simulink model "flightControlSystem"  (R2026b)
settings: Solver=ode3  StopTime=TFinal
PreLoadFcn:
  | InitVars;
  | definePX4ParamsBus;
undefined symbols (not defined in the file): control_power, DiscIntNeverNeededParam, init, MC_PITCHRATE_MAX, MC_ROLLRATE_MAX, MC_YAWRATE_MAX, PX4_Params_Default, SampleTime, timestamp
libraries: px4Utilslib x52, px4uORBlib x10, vrlib x8, aerolibutil x8, simulink x5, sharedutil x3, matrix_library x2, raspberrypiutilitieslib x2, px4Peripheralslib x2, sharedtransform x1, px4Sensorslib x1
(part 2 of 4)

== system flightControlSystem/MultiCopter Controller/Angular Rate Control/RatePID_Core ==
  note: rate_setpoint = P .* rate_error + rate_int - D .* angular_accel + FF .* rate_sp;
  angular_rate_measured_rads : Inport
  angular_rate_setpoint_rads : Inport  Port=2
  torque_sp_achieved : Inport  Port=3
  vehicle_landed : Inport  Port=4
  mixer_unallocated_torque : Inport  Port=5
  gain_P_MC_ROLLRATE_P : Inport  Port=6
  gain_I_MC_ROLLRATE_I : Inport  Port=7
  gain_D_MC_ROLLRATE_D : Inport  Port=8
  integral_limit_MC_RR_INT_LIM : Inport  Port=9
  dt_s : Inport  Port=10
  angular_accel_filtered_rads2 : Inport  Port=11
  gain_FF_MC_ROLLRATE_FF : Inport  Port=12
  rate_integral_state_prev : Inport  Port=13
  ActuatorSaturation_Detector : Subsystem
  Assignment : Assignment  DiagnosticForDimensions=Warning  IndexOptions=Index vector (dialog)  Indices=3  OutputSizes=1
  DSR_MC_YAW_TQ_CUTOFF : DataStoreRead  DataStoreName=PX4_Params  DataStoreElements=PX4_Params.MC_YAW_TQ_CUTOFF  IndexOptions=Index vector (dialog)  Indices=1  OutputSizes=1
  If_IsLanded : If  IfExpression=u1 ~=0
  Mul_Dterm_D_x_AngAccel : Product
  Mul_FFterm_FF_x_RateSP : Product
  Mul_Pterm_P_x_RateError : Product
  NOT_InvertLanded : Logic  Operator=NOT  IconShape=distinctive  AllPortsSameDT=off  OutDataTypeStr=boolean
  Reshape{1..2,7..11,13} (8 alike) : Reshape
  Selector : Selector  InputPortWidth=3  IndexOptions=Index vector (dialog)  Indices=3  OutputSizes=1
  Sub_RateError_sp_minus_meas : Sum  Inputs=+-
  Sum_PID_FF_TotalTorque : Sum  Inputs=++-+  AccumDataTypeStr=single
  YawTorqueLPF_v116 : MATLAB Function  TreatAsAtomicUnit=on
  rate_integral : Subsystem
  torque_setpoint_Nm : Outport
  rate_integral_state_next : Outport  Port=2
  wires:
  Reshape7/1 -> Mul_Pterm_P_x_RateError/2
  Reshape9/1 -> Mul_Dterm_D_x_AngAccel/1
  gain_FF_MC_ROLLRATE_FF/1 -> Reshape11/1  "ff"
  Mul_Pterm_P_x_RateError/1 -> Sum_PID_FF_TotalTorque/1
  vehicle_landed/1 -> NOT_InvertLanded/1
  angular_rate_setpoint_rads/1 -> Reshape2/1  "rate_sp"
  Sub_RateError_sp_minus_meas/1 -> Reshape7/1, rate_integral/8(rate_error_rads)  "rate_error"
  NOT_InvertLanded/1 -> If_IsLanded/1
  Reshape13/1 -> Sum_PID_FF_TotalTorque/2, rate_integral/9(integral_state_previous)
  Reshape2/1 -> Sub_RateError_sp_minus_meas/1, Mul_FFterm_FF_x_RateSP/2
  angular_rate_measured_rads/1 -> Reshape1/1
  rate_integral_state_prev/1 -> Reshape13/1  "rate_int"
  Reshape11/1 -> Mul_FFterm_FF_x_RateSP/1
  gain_P_MC_ROLLRATE_P/1 -> Reshape8/1  "Prop"
  gain_D_MC_ROLLRATE_D/1 -> Reshape9/1  "Der"
  angular_accel_filtered_rads2/1 -> Reshape10/1  "ang_accel"
  Mul_FFterm_FF_x_RateSP/1 -> Sum_PID_FF_TotalTorque/4
  Reshape8/1 -> Mul_Pterm_P_x_RateError/1
  Reshape10/1 -> Mul_Dterm_D_x_AngAccel/2
  Mul_Dterm_D_x_AngAccel/1 -> Sum_PID_FF_TotalTorque/3
  Reshape1/1 -> Sub_RateError_sp_minus_meas/2
  mixer_unallocated_torque/1 -> ActuatorSaturation_Detector/1(unallocated_torque_3x1)
  torque_sp_achieved/1 -> ActuatorSaturation_Detector/2(torque_setpoint_achieved)
  ActuatorSaturation_Detector/1(is_saturated_positive_3x1) -> rate_integral/1(mixer_saturated_positive)
  ActuatorSaturation_Detector/2(is_saturated_negative_3x1) -> rate_integral/2(mixer_saturated_negative)
  gain_I_MC_ROLLRATE_I/1 -> rate_integral/3(gain_I_per_axis)
  If_IsLanded/1 -> rate_integral/4(landed_reset_to_zero)
  If_IsLanded/2 -> rate_integral/5(airborne_update_integral)
  integral_limit_MC_RR_INT_LIM/1 -> rate_integral/6(integral_limit_symmetric)
  dt_s/1 -> YawTorqueLPF_v116/2(dt), rate_integral/7(dt_s)
  rate_integral/1(integral_state_updated) -> rate_integral_state_next/1
  Sum_PID_FF_TotalTorque/1 -> Selector/1, Assignment/1
  Selector/1 -> YawTorqueLPF_v116/1(yaw_torque)
  YawTorqueLPF_v116/1(yaw_torque_filt) -> Assignment/2
  DSR_MC_YAW_TQ_CUTOFF/1 -> YawTorqueLPF_v116/3(MC_YAW_TQ_CUTOFF)
  Assignment/1 -> torque_setpoint_Nm/1

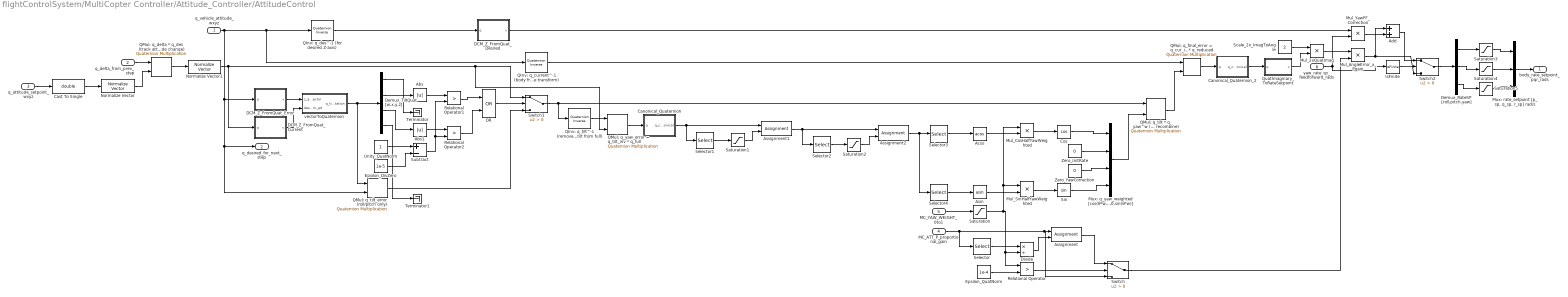
== system flightControlSystem/MultiCopter Controller/Attitude_Controller/AttitudeControl ==
  q_vehicle_attitude_wxyz : Inport
  q_delta_from_prev_step : Inport  Port=2
  q_attitude_setpoint_wxyz : Inport  Port=3
  MC_ATT_P_proportional_gain : Inport  Port=4
  MC_YAW_WEIGHT_0to1 : Inport  Port=5
  yaw_rate_sp_feedforward_rads : Inport  Port=6
  Abs : Abs  SaturateOnIntegerOverflow=off
  Abs1 : Abs  SaturateOnIntegerOverflow=off
  Acos : Trigonometry  Operator=acos
  Add : Sum
  Asin : Trigonometry  Operator=asin
  Assignment : Assignment  DiagnosticForDimensions=Warning  IndexOptions=Index vector (dialog)  Indices=3  OutputSizes=1  RuntimeRangeChecks=off
  Assignment1 : Assignment  DiagnosticForDimensions=Warning  IndexOptions=Index vector (dialog)  Indices=[1]  OutputSizes=1  RuntimeRangeChecks=off
  Assignment2 : Assignment  DiagnosticForDimensions=Warning  IndexOptions=Index vector (dialog)  Indices=[4]  OutputSizes=1  RuntimeRangeChecks=off
  Canonical_Quaternion : MATLAB Function  TreatAsAtomicUnit=on
  Canonical_Quaternion_2 : MATLAB Function  TreatAsAtomicUnit=on
  Cast To Single : DataTypeConversion  OutDataTypeStr=double  SaturateOnIntegerOverflow=off  RndMeth=Floor
  Cos : Trigonometry  Operator=cos
  DCM_Z_FromQuat_Current : MATLAB Function  TreatAsAtomicUnit=on
  DCM_Z_FromQuat_Desired : MATLAB Function  TreatAsAtomicUnit=on
  DCM_Z_FromQuat_Error : MATLAB Function  TreatAsAtomicUnit=on
  Demux_RateSP [roll,pitch,yaw] : Demux  Outputs=3
  Demux_TiltQuat [w,x,y,z] : Demux
  Divide : Product  Inputs=*/
  Epsilon_DivZero : Constant  Value=1e-5  SampleTime=-1
  Epsilon_QuatNorm : Constant  Value=1e-4  OutDataTypeStr=single  SampleTime=-1
  IsFinite : RelationalOperator  Operator=isFinite  OutDataTypeStr=boolean  RndMeth=Simplest  InputSameDT=off
  Mul_2xQuatImag : Product
  Mul_AngleError_x_Pgain : Product
  Mul_CosHalfYawWeighted : Product
  Mul_SinHalfYawWeighted : Product
  Mul_YawFF_Correction : Product
  Mux: q_yaw_weighted [cos(θ*w),0,0,sin(θ*w)] : Mux
  "Mux: rate_setpoint [p_sp, q_sp, r_sp] rad/s" : Mux  Inputs=3
  Normalize Vector : vrlib/Utilities/Normalize Vector  maxzero=0
  Normalize Vector1 : vrlib/Utilities/Normalize Vector  maxzero=0
  OR : Logic  Operator=OR  IconShape=distinctive  AllPortsSameDT=off  OutDataTypeStr=boolean
  QInv: q_current^-1 (body frame transform) : aerolibutil/Quaternion Inverse
  QInv: q_des^-1 (for desired Z-axis) : aerolibutil/Quaternion Inverse
  QInv: q_tilt^-1 (remove tilt from full) : aerolibutil/Quaternion Inverse
  QMul: q_delta * q_des (track attitude change) : aerolibutil/Quaternion Multiplication
  QMul: q_final_error = q_cur_inv * q_reduced : aerolibutil/Quaternion Multiplication
  QMul: q_tilt * q_yaw^w (weighted recombine) : aerolibutil/Quaternion Multiplication
  QMul: q_tilt_error (roll/pitch only) : aerolibutil/Quaternion Multiplication
  QMul: q_yaw_error = q_tilt_inv * q_full : aerolibutil/Quaternion Multiplication
  QuatImaginary_ToRateSetpoint : MATLAB Function  TreatAsAtomicUnit=on
  Relational Operator : RelationalOperator  Operator=>  OutDataTypeStr=boolean  RndMeth=Simplest  InputSameDT=off
  Relational Operator1 : RelationalOperator  Operator=>  OutDataTypeStr=boolean  RndMeth=Simplest  InputSameDT=off
  Relational Operator2 : RelationalOperator  Operator=>  OutDataTypeStr=boolean  RndMeth=Simplest  InputSameDT=off
  Saturation : Saturate  UpperLimit=1  LowerLimit=0
  Saturation1 : Saturate  UpperLimit=1  LowerLimit=-1
  Saturation2 : Saturate  UpperLimit=1  LowerLimit=-1
  Saturation3 : Saturate  UpperLimit=deg2rad(MC_ROLLRATE_MAX)  LowerLimit=-deg2rad(MC_ROLLRATE_MAX)
  Saturation4 : Saturate  UpperLimit=deg2rad(MC_PITCHRATE_MAX)  LowerLimit=-deg2rad(MC_PITCHRATE_MAX)
  Saturation5 : Saturate  UpperLimit=deg2rad(MC_YAWRATE_MAX)  LowerLimit=-deg2rad(MC_YAWRATE_MAX)
  Scale_2x_ImagToAngle : Constant  Value=2  SampleTime=-1
  Selector : Selector  InputPortWidth=3  IndexOptions=Index vector (dialog)  Indices=[3]  OutputSizes=1  RuntimeRangeChecks=off
  Selector1 : Selector  InputPortWidth=4  IndexOptions=Index vector (dialog)  Indices=[1]  OutputSizes=1  RuntimeRangeChecks=off
  Selector2 : Selector  InputPortWidth=4  IndexOptions=Index vector (dialog)  Indices=[4]  OutputSizes=1  RuntimeRangeChecks=off
  Selector3 : Selector  InputPortWidth=4  IndexOptions=Index vector (dialog)  Indices=[1]  OutputSizes=1  RuntimeRangeChecks=off
  Selector4 : Selector  InputPortWidth=4  IndexOptions=Index vector (dialog)  Indices=[4]  OutputSizes=1  RuntimeRangeChecks=off
  Sin : Trigonometry
  Subtract : Sum  Inputs=+-
  Switch : Switch  Criteria=u2 > Threshold  SaturateOnIntegerOverflow=off  InputSameDT=off
  Switch1 : Switch  Criteria=u2 > Threshold  SaturateOnIntegerOverflow=off  InputSameDT=off
  Switch2 : Switch  Criteria=u2 > Threshold  SaturateOnIntegerOverflow=off  InputSameDT=off
  Terminator : Terminator
  Terminator1 : Terminator
  Unity_QuatNorm : Constant  SampleTime=-1
  Zero_InitRate : Constant  Value=0  OutDataTypeStr=single  SampleTime=-1
  Zero_YawCorrection : Constant  Value=0  OutDataTypeStr=single  SampleTime=-1
  vectorToQuaternion : Subsystem
  body_rate_setpoint_pqr_rads : Outport
  q_desired_for_next_step : Outport  Port=2
  wires:
  MC_ATT_P_proportional_gain/1 -> Switch/3, Assignment/1, Selector/1
  Demux_TiltQuat [w,x,y,z]/3 -> Abs1/1
  q_attitude_setpoint_wxyz/1 -> Cast To Single/1
  q_vehicle_attitude_wxyz/1 -> QMul: q_tilt_error (roll/pitch only)/2, q_desired_for_next_step/1, DCM_Z_FromQuat_Error/1(q), QInv: q_current^-1 (body frame transform)/1, QInv: q_des^-1 (for desired Z-axis)/1
  Mul_YawFF_Correction/1 -> Add/2
  Epsilon_DivZero/1 -> Subtract/2
  DCM_Z_FromQuat_Current/1(v) -> vectorToQuaternion/2(desired_z_axis_from_qd)
  q_delta_from_prev_step/1 -> QMul: q_delta * q_des (track attitude change)/1
  Cast To Single/1 -> Normalize Vector/1
  Saturation2/1 -> Assignment2/2
  Switch1/1 -> QMul: q_tilt * q_yaw^w (weighted recombine)/1, QInv: q_tilt^-1 (remove tilt from full)/1
  Normalize Vector/1 -> QMul: q_delta * q_des (track attitude change)/2
  DCM_Z_FromQuat_Desired/1(v) -> Mul_YawFF_Correction/1
  QMul: q_delta * q_des (track attitude change)/1 -> Normalize Vector1/1
  Normalize Vector1/1 -> QMul: q_yaw_error = q_tilt_inv * q_full/2, Switch1/1, DCM_Z_FromQuat_Current/1(q)
  DCM_Z_FromQuat_Error/1(v) -> vectorToQuaternion/1(z_axis_unit_vector)
  QInv: q_des^-1 (for desired Z-axis)/1 -> DCM_Z_FromQuat_Desired/1(q)
  vectorToQuaternion/1(q_tilt_rotation) -> QMul: q_tilt_error (roll/pitch only)/1, Demux_TiltQuat [w,x,y,z]/1
  Demux_TiltQuat [w,x,y,z]/1 -> Terminator/1
  Canonical_Quaternion_2/1(q_canonical) -> QuatImaginary_ToRateSetpoint/1(q)
  Selector3/1 -> Acos/1
  Selector2/1 -> Saturation2/1
  Demux_TiltQuat [w,x,y,z]/2 -> Abs/1
  Demux_TiltQuat [w,x,y,z]/4 -> Terminator1/1
  Epsilon_QuatNorm/1 -> Relational Operator/2
  Unity_QuatNorm/1 -> Subtract/1
  QMul: q_tilt_error (roll/pitch only)/1 -> Switch1/3
  Abs/1 -> Relational Operator1/1
  Mux: q_yaw_weighted [cos(θ*w),0,0,sin(θ*w)]/1 -> QMul: q_tilt * q_yaw^w (weighted recombine)/2
  Relational Operator2/1 -> OR/2
  Abs1/1 -> Relational Operator2/1
  Subtract/1 -> Relational Operator1/2, Relational Operator2/2
  Relational Operator1/1 -> OR/1
  OR/1 -> Switch1/2
  QInv: q_current^-1 (body frame transform)/1 -> QMul: q_final_error = q_cur_inv * q_reduced/1
  QInv: q_tilt^-1 (remove tilt from full)/1 -> QMul: q_yaw_error = q_tilt_inv * q_full/1
  Selector/1 -> Divide/1
  QMul: q_yaw_error = q_tilt_inv * q_full/1 -> Canonical_Quaternion/1(q)
  QMul: q_final_error = q_cur_inv * q_reduced/1 -> Canonical_Quaternion_2/1(q)
  Canonical_Quaternion/1(q_canonical) -> Assignment1/1, Selector1/1
  Selector1/1 -> Saturation1/1
  Cos/1 -> Mux: q_yaw_weighted [cos(θ*w),0,0,sin(θ*w)]/1
  Mul_SinHalfYawWeighted/1 -> Sin/1
  Saturation1/1 -> Assignment1/2
  Assignment1/1 -> Assignment2/1, Selector2/1
  Assignment2/1 -> Selector3/1, Selector4/1
  yaw_rate_sp_feedforward_rads/1 -> IsFinite/1, Mul_YawFF_Correction/2
  Zero_InitRate/1 -> Mux: q_yaw_weighted [cos(θ*w),0,0,sin(θ*w)]/2
  MC_YAW_WEIGHT_0to1/1 -> Saturation/1
  Selector4/1 -> Asin/1
  Acos/1 -> Mul_CosHalfYawWeighted/2
  Assignment/1 -> Switch/1
  Asin/1 -> Mul_SinHalfYawWeighted/2
  Saturation/1 -> Divide/2, Relational Operator/1, Mul_SinHalfYawWeighted/1, Mul_CosHalfYawWeighted/1
  Mul_CosHalfYawWeighted/1 -> Cos/1
  Divide/1 -> Assignment/2
  Relational Operator/1 -> Switch/2
  Sin/1 -> Mux: q_yaw_weighted [cos(θ*w),0,0,sin(θ*w)]/4
  Zero_YawCorrection/1 -> Mux: q_yaw_weighted [cos(θ*w),0,0,sin(θ*w)]/3
  Switch/1 -> Mul_AngleError_x_Pgain/2
  QMul: q_tilt * q_yaw^w (weighted recombine)/1 -> QMul: q_final_error = q_cur_inv * q_reduced/2
  Scale_2x_ImagToAngle/1 -> Mul_2xQuatImag/1
  QuatImaginary_ToRateSetpoint/1(v) -> Mul_2xQuatImag/2
  Mul_2xQuatImag/1 -> Mul_AngleError_x_Pgain/1
  Mul_AngleError_x_Pgain/1 -> Switch2/3, Add/1
  Add/1 -> Switch2/1
  IsFinite/1 -> Switch2/2
  Switch2/1 -> Demux_RateSP [roll,pitch,yaw]/1
  Demux_RateSP [roll,pitch,yaw]/1 -> Saturation3/1
  Demux_RateSP [roll,pitch,yaw]/2 -> Saturation4/1
  Demux_RateSP [roll,pitch,yaw]/3 -> Saturation5/1
  Saturation3/1 -> "Mux: rate_setpoint [p_sp, q_sp, r_sp] rad/s"/1
  Saturation4/1 -> "Mux: rate_setpoint [p_sp, q_sp, r_sp] rad/s"/2
  Saturation5/1 -> "Mux: rate_setpoint [p_sp, q_sp, r_sp] rad/s"/3
  "Mux: rate_setpoint [p_sp, q_sp, r_sp] rad/s"/1 -> body_rate_setpoint_pqr_rads/1

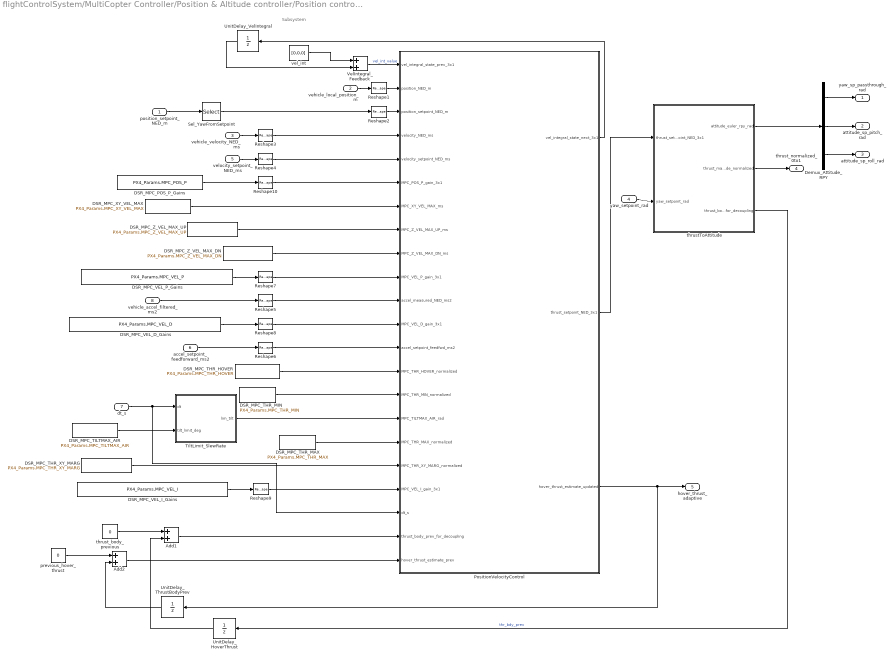
== system flightControlSystem/MultiCopter Controller/Position & Altitude controller/Position controller ==
  note: Subsystem
  position_setpoint_NED_m : Inport
  vehicle_local_position_m : Inport  Port=2
  vehicle_velocity_NED_ms : Inport  Port=3
  yaw_setpoint_rad : Inport  Port=4
  velocity_setpoint_NED_ms : Inport  Port=5
  accel_setpoint_feedforward_ms2 : Inport  Port=6
  dt_s : Inport  Port=7
  vehicle_accel_filtered_ms2 : Inport  Port=8
  Add1 : Sum
  Add2 : Sum
  DSR_MPC_POS_P_Gains : DataStoreRead  DataStoreName=PX4_Params  DataStoreElements=PX4_Params.MPC_POS_P  IndexOptions=Index vector (dialog)  Indices=1  OutputSizes=1
  DSR_MPC_THR_HOVER : DataStoreRead  DataStoreName=PX4_Params  DataStoreElements=PX4_Params.MPC_THR_HOVER  IndexOptions=Index vector (dialog)  Indices=1  OutputSizes=1
  DSR_MPC_THR_MAX : DataStoreRead  DataStoreName=PX4_Params  DataStoreElements=PX4_Params.MPC_THR_MAX  IndexOptions=Index vector (dialog)  Indices=1  OutputSizes=1
  DSR_MPC_THR_MIN : DataStoreRead  DataStoreName=PX4_Params  DataStoreElements=PX4_Params.MPC_THR_MIN  IndexOptions=Index vector (dialog)  Indices=1  OutputSizes=1
  DSR_MPC_THR_XY_MARG : DataStoreRead  DataStoreName=PX4_Params  DataStoreElements=PX4_Params.MPC_THR_XY_MARG  IndexOptions=Index vector (dialog)  Indices=1  OutputSizes=1
  DSR_MPC_TILTMAX_AIR : DataStoreRead  DataStoreName=PX4_Params  DataStoreElements=PX4_Params.MPC_TILTMAX_AIR  IndexOptions=Index vector (dialog)  Indices=1  OutputSizes=1
  DSR_MPC_VEL_D_Gains : DataStoreRead  DataStoreName=PX4_Params  DataStoreElements=PX4_Params.MPC_VEL_D  IndexOptions=Index vector (dialog)  Indices=1  OutputSizes=1
  DSR_MPC_VEL_I_Gains : DataStoreRead  DataStoreName=PX4_Params  DataStoreElements=PX4_Params.MPC_VEL_I  IndexOptions=Index vector (dialog)  Indices=1  OutputSizes=1
  DSR_MPC_VEL_P_Gains : DataStoreRead  DataStoreName=PX4_Params  DataStoreElements=PX4_Params.MPC_VEL_P  IndexOptions=Index vector (dialog)  Indices=1  OutputSizes=1
  DSR_MPC_XY_VEL_MAX : DataStoreRead  DataStoreName=PX4_Params  DataStoreElements=PX4_Params.MPC_XY_VEL_MAX  IndexOptions=Index vector (dialog)  Indices=1  OutputSizes=1
  DSR_MPC_Z_VEL_MAX_DN : DataStoreRead  DataStoreName=PX4_Params  DataStoreElements=PX4_Params.MPC_Z_VEL_MAX_DN  IndexOptions=Index vector (dialog)  Indices=1  OutputSizes=1
  DSR_MPC_Z_VEL_MAX_UP : DataStoreRead  DataStoreName=PX4_Params  DataStoreElements=PX4_Params.MPC_Z_VEL_MAX_UP  IndexOptions=Index vector (dialog)  Indices=1  OutputSizes=1
  Demux_Attitude_RPY : Demux  Outputs=3
  PositionVelocityControl : Subsystem
  Reshape{1..10} (10 alike) : Reshape
  Sel_YawFromSetpoint : Selector  InputPortWidth=4  IndexOptions=Index vector (dialog)  Indices=[1:3]  OutputSizes=1  RuntimeRangeChecks=off
  TiltLimit_SlewRate : MATLAB Function  TreatAsAtomicUnit=on
  UnitDelay_HoverThrust : UnitDelay  SampleTime=-1
  UnitDelay_ThrustBodyPrev : UnitDelay  SampleTime=-1
  UnitDelay_VelIntegral : UnitDelay  InitialCondition=[0; 0; 0]  SampleTime=-1
  VelIntegral_Feedback : Sum
  previous_hover_thrust : Constant  Value=0  OutDataTypeStr=single  SampleTime=-1
  thrustToAttitude : Subsystem
  thrust_body_previous : Constant  Value=0  OutDataTypeStr=single  SampleTime=-1
  vel_int : Constant  Value=[0,0,0]  OutDataTypeStr=single  SampleTime=-1
  yaw_sp_passthrough_rad : Outport
  attitude_sp_pitch_rad : Outport  Port=2
  attitude_sp_roll_rad : Outport  Port=3
  thrust_normalized_0to1 : Outport  Port=4
  hover_thrust_adaptive : Outport  Port=5
  wires:
  thrustToAttitude/1(attitude_euler_rpy_rad) -> Demux_Attitude_RPY/1
  previous_hover_thrust/1 -> Add2/1
  vel_int/1 -> VelIntegral_Feedback/1
  thrust_body_previous/1 -> Add1/1
  position_setpoint_NED_m/1 -> Sel_YawFromSetpoint/1
  UnitDelay_HoverThrust/1 -> Add1/2
  DSR_MPC_TILTMAX_AIR/1 -> TiltLimit_SlewRate/2(tilt_limit_deg)
  UnitDelay_VelIntegral/1 -> VelIntegral_Feedback/2
  UnitDelay_ThrustBodyPrev/1 -> Add2/2
  Demux_Attitude_RPY/1 -> yaw_sp_passthrough_rad/1
  thrustToAttitude/2(thrust_magnitude_normalized) -> thrust_normalized_0to1/1
  PositionVelocityControl/3(hover_thrust_estimate_updated) -> UnitDelay_ThrustBodyPrev/1, hover_thrust_adaptive/1
  PositionVelocityControl/1(vel_integral_state_next_3x1) -> UnitDelay_VelIntegral/1
  Demux_Attitude_RPY/3 -> attitude_sp_roll_rad/1
  Demux_Attitude_RPY/2 -> attitude_sp_pitch_rad/1
  thrustToAttitude/3(thrust_body_frame_for_decoupling) -> UnitDelay_HoverThrust/1  "thr_bdy_prev"
  PositionVelocityControl/2(thrust_setpoint_NED_3x1) -> thrustToAttitude/1(thrust_setpoint_NED_3x1)
  Reshape9/1 -> PositionVelocityControl/19(MPC_VEL_I_gain_3x1)
  DSR_MPC_THR_XY_MARG/1 -> PositionVelocityControl/18(MPC_THR_XY_MARG_normalized)
  DSR_MPC_THR_MAX/1 -> PositionVelocityControl/17(MPC_THR_MAX_normalized)
  dt_s/1 -> TiltLimit_SlewRate/1(dt), PositionVelocityControl/20(dt_s)
  DSR_MPC_THR_MIN/1 -> PositionVelocityControl/15(MPC_THR_MIN_normalized)
  DSR_MPC_THR_HOVER/1 -> PositionVelocityControl/14(MPC_THR_HOVER_normalized)
  Reshape6/1 -> PositionVelocityControl/13(accel_setpoint_feedfwd_ms2)
  Reshape8/1 -> PositionVelocityControl/12(MPC_VEL_D_gain_3x1)
  Reshape7/1 -> PositionVelocityControl/10(MPC_VEL_P_gain_3x1)
  DSR_MPC_Z_VEL_MAX_UP/1 -> PositionVelocityControl/8(MPC_Z_VEL_MAX_UP_ms)
  Reshape10/1 -> PositionVelocityControl/6(MPC_POS_P_gain_3x1)
  Reshape4/1 -> PositionVelocityControl/5(velocity_setpoint_NED_ms)
  Reshape5/1 -> PositionVelocityControl/11(accel_measured_NED_ms2)
  Reshape3/1 -> PositionVelocityControl/4(velocity_NED_ms)
  Reshape2/1 -> PositionVelocityControl/3(position_setpoint_NED_m)
  accel_setpoint_feedforward_ms2/1 -> Reshape6/1
  DSR_MPC_XY_VEL_MAX/1 -> PositionVelocityControl/7(MPC_XY_VEL_MAX_ms)
  DSR_MPC_VEL_P_Gains/1 -> Reshape7/1
  yaw_setpoint_rad/1 -> thrustToAttitude/2(yaw_setpoint_rad)
  DSR_MPC_POS_P_Gains/1 -> Reshape10/1
  Reshape1/1 -> PositionVelocityControl/2(position_NED_m)
  DSR_MPC_Z_VEL_MAX_DN/1 -> PositionVelocityControl/9(MPC_Z_VEL_MAX_DN_ms)
  vehicle_accel_filtered_ms2/1 -> Reshape5/1
  velocity_setpoint_NED_ms/1 -> Reshape4/1
  vehicle_velocity_NED_ms/1 -> Reshape3/1
  Sel_YawFromSetpoint/1 -> Reshape2/1
  vehicle_local_position_m/1 -> Reshape1/1
  DSR_MPC_VEL_D_Gains/1 -> Reshape8/1
  DSR_MPC_VEL_I_Gains/1 -> Reshape9/1
  TiltLimit_SlewRate/1(lim_tilt) -> PositionVelocityControl/16(MPC_TILTMAX_AIR_rad)
  VelIntegral_Feedback/1 -> PositionVelocityControl/1(vel_integral_state_prev_3x1)  "vel_int_value"
  Add1/1 -> PositionVelocityControl/21(thrust_body_prev_for_decoupling)
  Add2/1 -> PositionVelocityControl/22(hover_thrust_estimate_prev)

== system flightControlSystem/ParamUpdate/HW_ParamUpdate/ReadParams_OnUpdate ==
  Enable : EnablePort
  AttitudeCtrl_Params : Subsystem
  BusCreator_Params : BusCreator  Inputs=30  OutDataTypeStr=Bus: PX4_Params_Bus
  Estimator_Params : Subsystem
  LandingLogic_Params : Subsystem
  PositionCtrl_Params : Subsystem
  RateCtrl_Params : Subsystem
  Signal Conversion : SignalConversion  ConversionOutput=Nonvirtual bus  OverrideOpt=off
  Write_PX4_Params : DataStoreWrite  DataStoreName=PX4_Params  IndexOptions=Index vector (dialog)  Indices=1  OutputSizes=1
  wires:
  RateCtrl_Params/4(MC_RATE_FF) -> BusCreator_Params/19  "MC_RATE_FF"
  PositionCtrl_Params/8(MPC_THR_XY_MARG) -> BusCreator_Params/8  "MPC_THR_XY_MARG"
  Estimator_Params/2(EST_NF_FRQ) -> BusCreator_Params/29  "EST_NF_FRQ"
  LandingLogic_Params/6(MPC_Z_VEL_MAX_DN_LAND) -> BusCreator_Params/27  "MPC_Z_VEL_MAX_DN_LAND"
  PositionCtrl_Params/2(MPC_VEL_P) -> BusCreator_Params/2  "MPC_VEL_P"
  PositionCtrl_Params/1(MPC_POS_P) -> BusCreator_Params/1  "MPC_POS_P"
  PositionCtrl_Params/5(MPC_THR_HOVER) -> BusCreator_Params/5  "MPC_THR_HOVER"
  PositionCtrl_Params/11(MPC_Z_VEL_MAX_UP) -> BusCreator_Params/11  "MPC_Z_VEL_MAX_UP"
  Estimator_Params/1(MPC_VELD_LP) -> BusCreator_Params/28  "MPC_VELD_LP"
  AttitudeCtrl_Params/2(MC_YAW_WEIGHT) -> BusCreator_Params/15  "MC_YAW_WEIGHT"
  PositionCtrl_Params/3(MPC_VEL_I) -> BusCreator_Params/3  "MPC_VEL_I"
  PositionCtrl_Params/6(MPC_THR_MAX) -> BusCreator_Params/6  "MPC_THR_MAX"
  Estimator_Params/3(EST_NF_BW) -> BusCreator_Params/30  "EST_NF_BW"
  Signal Conversion/1 -> Write_PX4_Params/1
  PositionCtrl_Params/4(MPC_VEL_D) -> BusCreator_Params/4  "MPC_VEL_D"
  BusCreator_Params/1 -> Signal Conversion/1
  LandingLogic_Params/1(MPC_LAND_ALT1) -> BusCreator_Params/22  "MPC_LAND_ALT1"
  LandingLogic_Params/2(MPC_LAND_ALT2) -> BusCreator_Params/23  "MPC_LAND_ALT2"
  PositionCtrl_Params/7(MPC_THR_MIN) -> BusCreator_Params/7  "MPC_THR_MIN"
  AttitudeCtrl_Params/1(MC_ATT_P) -> BusCreator_Params/14  "MC_ATT_P"
  LandingLogic_Params/3(MPC_LAND_ALT3) -> BusCreator_Params/24  "MPC_LAND_ALT3"
  RateCtrl_Params/2(MC_RATE_I) -> BusCreator_Params/17  "MC_RATE_I"
  LandingLogic_Params/4(MPC_LAND_SPEED) -> BusCreator_Params/25  "MPC_LAND_SPEED"
  LandingLogic_Params/5(MPC_LAND_CRWL) -> BusCreator_Params/26  "MPC_LAND_CRWL"
  PositionCtrl_Params/9(MPC_TILTMAX_AIR) -> BusCreator_Params/9  "MPC_TILTMAX_AIR"
  RateCtrl_Params/5(MC_RATE_INT_LIM) -> BusCreator_Params/20  "MC_RATE_INT_LIM"
  RateCtrl_Params/1(MC_RATE_P) -> BusCreator_Params/16  "MC_RATE_P"
  RateCtrl_Params/6(MC_YAW_TQ_CUTOFF) -> BusCreator_Params/21  "MC_YAW_TQ_CUTOFF"
  PositionCtrl_Params/10(MPC_XY_VEL_MAX) -> BusCreator_Params/10  "MPC_XY_VEL_MAX"
  PositionCtrl_Params/12(MPC_Z_VEL_MAX_DN) -> BusCreator_Params/12  "MPC_Z_VEL_MAX_DN"
  RateCtrl_Params/3(MC_RATE_D) -> BusCreator_Params/18  "MC_RATE_D"
  PositionCtrl_Params/13(MPC_ACC_DECOUPLE) -> BusCreator_Params/13  "MPC_ACC_DECOUPLE"

== system flightControlSystem/SetpointManager/Set target Position/Landing Logic ==
  Current_Pos : Inport
  land_trigger : Inport  Port=2
  DSR_MPC_LAND_ALT1 : DataStoreRead  DataStoreName=PX4_Params  DataStoreElements=PX4_Params.MPC_LAND_ALT1  IndexOptions=Index vector (dialog)  Indices=1  OutputSizes=1
  DSR_MPC_LAND_ALT2 : DataStoreRead  DataStoreName=PX4_Params  DataStoreElements=PX4_Params.MPC_LAND_ALT2  IndexOptions=Index vector (dialog)  Indices=1  OutputSizes=1
  DSR_MPC_LAND_ALT3 : DataStoreRead  DataStoreName=PX4_Params  DataStoreElements=PX4_Params.MPC_LAND_ALT3  IndexOptions=Index vector (dialog)  Indices=1  OutputSizes=1
  DSR_MPC_LAND_CRWL : DataStoreRead  DataStoreName=PX4_Params  DataStoreElements=PX4_Params.MPC_LAND_CRWL  IndexOptions=Index vector (dialog)  Indices=1  OutputSizes=1
  DSR_MPC_LAND_SPEED : DataStoreRead  DataStoreName=PX4_Params  DataStoreElements=PX4_Params.MPC_LAND_SPEED  IndexOptions=Index vector (dialog)  Indices=1  OutputSizes=1
  DSR_MPC_Z_VEL_MAX_DN : DataStoreRead  DataStoreName=PX4_Params  DataStoreElements=PX4_Params.MPC_Z_VEL_MAX_DN_LAND  IndexOptions=Index vector (dialog)  Indices=1  OutputSizes=1
  PX4 Landing Logic : MATLAB Function  TreatAsAtomicUnit=on
  Selector1 : Selector  InputPortWidth=5  IndexOptions=Index vector (dialog)  Indices=[1:4]  OutputSizes=1  RuntimeRangeChecks=off
  pos_sp : Outport
  vel_sp : Outport  Port=2
  acc_sp : Outport  Port=3
  wires:
  Current_Pos/1 -> Selector1/1
  DSR_MPC_LAND_CRWL/1 -> PX4 Landing Logic/4(MPC_LAND_CRWL_in)
  Selector1/1 -> PX4 Landing Logic/2(states)
  DSR_MPC_LAND_SPEED/1 -> PX4 Landing Logic/3(MPC_LAND_SPEED_in)
  DSR_MPC_LAND_ALT1/1 -> PX4 Landing Logic/5(MPC_LAND_ALT1_in)
  DSR_MPC_Z_VEL_MAX_DN/1 -> PX4 Landing Logic/8(MPC_Z_VEL_MAX_DN_in)
  DSR_MPC_LAND_ALT2/1 -> PX4 Landing Logic/6(MPC_LAND_ALT2_in)
  DSR_MPC_LAND_ALT3/1 -> PX4 Landing Logic/7(MPC_LAND_ALT3_in)
  PX4 Landing Logic/1(pos_sp) -> pos_sp/1
  PX4 Landing Logic/2(vel_sp) -> vel_sp/1
  PX4 Landing Logic/3(acc_sp) -> acc_sp/1
  land_trigger/1 -> PX4 Landing Logic/1(land_trigger)

== system flightControlSystem/SetpointManager/Set target Position/Logger ==
  DesiredPosition : Inport
  DesiredVelocity : Inport  Port=2
  DesiredAcceleration : Inport  Port=3
  States : Inport  Port=4
  Cast To Single{,1..13} (14 alike) : DataTypeConversion  OutDataTypeStr=single  SaturateOnIntegerOverflow=off  RndMeth=Floor
  Demux : Demux
  Demux1 : Demux
  Demux2 : Demux  Outputs=3
  Demux3 : Demux  Outputs=3
  PX4 ULog : px4Utilslib/PX4 ULog  Commented=on  uORBMsg=FlightChecks
  Rate Transition : RateTransition
  Rate Transition2 : RateTransition
  Selector : Selector  InputPortWidth=5  IndexOptions=Index vector (dialog)  Indices=[1:4]  OutputSizes=1
  wires:
  Cast To Single2/1 -> ?
  Demux/1 -> Cast To Single/1
  Cast To Single5/1 -> PX4 ULog/2
  Rate Transition2/1 -> Demux1/1
  Demux1/3 -> Cast To Single6/1
  Cast To Single7/1 -> PX4 ULog/4
  Demux1/1 -> Cast To Single4/1
  Rate Transition/1 -> Demux/1
  Cast To Single6/1 -> PX4 ULog/3
  DesiredPosition/1 -> Rate Transition2/1
  DesiredAcceleration/1 -> Demux3/1
  Demux1/2 -> Cast To Single5/1
  Demux2/1 -> Cast To Single8/1
  Cast To Single4/1 -> PX4 ULog/1
  Demux3/2 -> Cast To Single12/1
  Demux/2 -> Cast To Single1/1
  Demux1/4 -> Cast To Single7/1
  Cast To Single8/1 -> ?
  Demux2/2 -> Cast To Single9/1
  Cast To Single9/1 -> ?
  Cast To Single10/1 -> ?
  Demux2/3 -> Cast To Single10/1
  Demux3/1 -> Cast To Single11/1
  Cast To Single11/1 -> ?
  Cast To Single13/1 -> ?
  Cast To Single12/1 -> ?
  Demux3/3 -> Cast To Single13/1
  Cast To Single/1 -> ?
  Cast To Single1/1 -> ?
  Demux/3 -> Cast To Single2/1
  Demux/4 -> Cast To Single3/1
  Cast To Single3/1 -> ?
  States/1 -> Selector/1
  DesiredVelocity/1 -> Demux2/1
  Selector/1 -> Rate Transition/1

== system flightControlSystem/SetpointManager/Set target Position/RC Failsafe Signal ==
  note: Channel 7 - RC Flysky
      | Channel 7 - Dexi Radiomaster
  Constant1 : Constant  SampleTime=-1
  MATLAB Function : MATLAB Function  TreatAsAtomicUnit=on
  Radio Control Transmitter1 : px4Sensorslib/Radio Control Transmitter  channel1=off  channel2=off  channel3=off  channel4=off  channel5=off  channel6=off  channel7=on  channel8=off  channel_count=off  rssi=on  rc_input_source=off  timestamp_last_signal=off  time_stamp=off  sampleTime=1/250  BlockingMode=off  BlockTimeout=5
  Rate Transition3 : RateTransition
  Switch1 : Switch  Criteria=u2 ~= 0  SaturateOnIntegerOverflow=off  InputSameDT=off
  Unit Delay : UnitDelay  SampleTime=-1
  Land_Trigger : Outport
  wires:
  Constant1/1 -> Switch1/1
  Radio Control Transmitter1/3 -> MATLAB Function/3(RSSI)
  Radio Control Transmitter1/2 -> MATLAB Function/2(ch7)
  Radio Control Transmitter1/1 -> MATLAB Function/1(status)
  MATLAB Function/1(out) -> Rate Transition3/1
  Rate Transition3/1 -> Switch1/2
  Unit Delay/1 -> Switch1/3
  Switch1/1 -> Unit Delay/1, Land_Trigger/1

== system flightControlSystem/SetpointManager/Set target Position/Setpoints Selector ==
  Land_Pos : Inport
  Land_Vel : Inport  Port=2
  Land_Acc : Inport  Port=3
  LandTrigger : Inport  Port=4
  Des_Pos : Inport  Port=5
  Des_Vel : Inport  Port=6
  Des_Acc : Inport  Port=7
  Acc Switch : Switch  Criteria=u2 > Threshold  SaturateOnIntegerOverflow=off  InputSameDT=off
  Rate Transition2 : RateTransition
  Rate Transition4 : RateTransition
  Rate Transition5 : RateTransition
  Reshape : Reshape
  Switch : Switch  Criteria=u2 > Threshold  SaturateOnIntegerOverflow=off  InputSameDT=off
  Vel Switch : Switch  Criteria=u2 > Threshold  SaturateOnIntegerOverflow=off  InputSameDT=off
  des_pos : Outport
  des_vel : Outport  Port=2
  des_acc : Outport  Port=3
  wires:
  Land_Acc/1 -> Acc Switch/1
  Acc Switch/1 -> Rate Transition5/1
  Reshape/1 -> Switch/1
  LandTrigger/1 -> Vel Switch/2, Switch/2, Acc Switch/2
  Switch/1 -> Rate Transition2/1
  Vel Switch/1 -> Rate Transition4/1
  Land_Pos/1 -> Reshape/1
  Land_Vel/1 -> Vel Switch/1
  Rate Transition2/1 -> des_pos/1
  Des_Pos/1 -> Switch/3
  Rate Transition4/1 -> des_vel/1
  Des_Vel/1 -> Vel Switch/3
  Rate Transition5/1 -> des_acc/1
  Des_Acc/1 -> Acc Switch/3

== system flightControlSystem/SetpointManager/Set target Position/Setpoints from Perception Module ==
  CurrentPosition : Inport
  AND : Logic  IconShape=distinctive  AllPortsSameDT=off  OutDataTypeStr=boolean
  Cast To Boolean : DataTypeConversion  OutDataTypeStr=boolean  SaturateOnIntegerOverflow=off  RndMeth=Floor
  Cast To Double : DataTypeConversion  OutDataTypeStr=double  SaturateOnIntegerOverflow=off  RndMeth=Floor
  Compare To Constant1 : simulink/Logic and Bit Operations/Compare To Constant  relop===  const=222  OutDataTypeStr=boolean
  Demux : Demux  Outputs=11
  Enabled Subsystem : Subsystem  TreatAsAtomicUnit=on
  Mux : Mux
  Mux1 : Mux  Inputs=3
  Mux2 : Mux  Inputs=3
  Protocol Decoder : raspberrypiutilitieslib/Protocol Decoder  IsParseCSV=off  Header=[134]  FieldTable={ 'Field1', '11', 'single', 'Little endian' }  IsVariableSizeLastField=off  MaxVariableSizeFieldLength=[]  IsChecksumRequired=off  ChecksumAlgorithm=XOR of bytes  ChecksumSize=[]  TerminatorOption=<none>  CustomTerminatorVal=[]  IsInputLengthAvailable=off
  Selector : Selector  InputPortWidth=5  IndexOptions=Index vector (dialog)  Indices=[5]  OutputSizes=1  RuntimeRangeChecks=off
  Serial Receive : px4Peripheralslib/Serial Receive  SCIModule=/dev/ttyACM0  DataType=uint8  DataLength=45  OutputStatus=on  SampleTime=1/10  BlockingMode=off  PartialData=on  Timeout=5
  Switch2 : Switch  Criteria=u2 > Threshold  SaturateOnIntegerOverflow=off  InputSameDT=off
  Terminator : Terminator
  Terminator1 : Terminator
  Unit Delay : UnitDelay  SampleTime=-1
  des Position : Outport
  desired Velocity : Outport  Port=2
  desired Acceleration : Outport  Port=3
  wires:
  Demux/1 -> Mux/1
  Demux/3 -> Mux/3
  Demux/11 -> Compare To Constant1/1
  AND/1 -> Enabled Subsystem/Enable
  Demux/6 -> Mux1/2
  Demux/10 -> Mux2/3
  Selector/1 -> Cast To Boolean/1
  Compare To Constant1/1 -> AND/2, Switch2/2
  Protocol Decoder/1 -> Cast To Double/1
  Cast To Double/1 -> Demux/1
  Demux/2 -> Mux/2
  Demux/9 -> Mux2/2
  Protocol Decoder/2 -> Terminator/1
  Cast To Boolean/1 -> AND/1
  Demux/8 -> Mux2/1
  Demux/5 -> Mux1/1
  Serial Receive/1 -> Protocol Decoder/1
  Mux/1 -> Switch2/1
  Unit Delay/1 -> Switch2/3
  Switch2/1 -> des Position/1, Unit Delay/1
  CurrentPosition/1 -> Selector/1, Enabled Subsystem/1(CurrentPosition)
  Demux/4 -> Mux/4
  Demux/7 -> Mux1/3
  Serial Receive/2 -> Terminator1/1
  Mux1/1 -> desired Velocity/1
  Mux2/1 -> desired Acceleration/1

== system flightControlSystem/SetpointManager/Simulation Set target Position/Landing Logic ==
  Current_Pos : Inport
  land_trigger : Inport  Port=2
  DSR_MPC_LAND_ALT1_const : DataStoreRead  DataStoreName=PX4_Params  DataStoreElements=PX4_Params.MPC_LAND_ALT1  IndexOptions=Index vector (dialog)  Indices=1  OutputSizes=1
  DSR_MPC_LAND_ALT2_const : DataStoreRead  DataStoreName=PX4_Params  DataStoreElements=PX4_Params.MPC_LAND_ALT2  IndexOptions=Index vector (dialog)  Indices=1  OutputSizes=1
  DSR_MPC_LAND_ALT3_const : DataStoreRead  DataStoreName=PX4_Params  DataStoreElements=PX4_Params.MPC_LAND_ALT3  IndexOptions=Index vector (dialog)  Indices=1  OutputSizes=1
  DSR_MPC_LAND_CRWL_const : DataStoreRead  DataStoreName=PX4_Params  DataStoreElements=PX4_Params.MPC_LAND_CRWL  IndexOptions=Index vector (dialog)  Indices=1  OutputSizes=1
  DSR_MPC_LAND_SPEED_const : DataStoreRead  DataStoreName=PX4_Params  DataStoreElements=PX4_Params.MPC_LAND_SPEED  IndexOptions=Index vector (dialog)  Indices=1  OutputSizes=1
  DSR_MPC_Z_VEL_MAX_DN_const : DataStoreRead  DataStoreName=PX4_Params  DataStoreElements=PX4_Params.MPC_Z_VEL_MAX_DN_LAND  IndexOptions=Index vector (dialog)  Indices=1  OutputSizes=1
  PX4 Landing Logic : MATLAB Function  TreatAsAtomicUnit=on
  Selector1 : Selector  InputPortWidth=5  IndexOptions=Index vector (dialog)  Indices=[1:4]  OutputSizes=1  RuntimeRangeChecks=off
  pos_sp : Outport
  vel_sp : Outport  Port=2
  acc_sp : Outport  Port=3
  wires:
  Current_Pos/1 -> Selector1/1
  DSR_MPC_LAND_CRWL_const/1 -> PX4 Landing Logic/4(MPC_LAND_CRWL_in)
  Selector1/1 -> PX4 Landing Logic/2(states)
  DSR_MPC_LAND_SPEED_const/1 -> PX4 Landing Logic/3(MPC_LAND_SPEED_in)
  DSR_MPC_LAND_ALT1_const/1 -> PX4 Landing Logic/5(MPC_LAND_ALT1_in)
  DSR_MPC_Z_VEL_MAX_DN_const/1 -> PX4 Landing Logic/8(MPC_Z_VEL_MAX_DN_in)
  DSR_MPC_LAND_ALT2_const/1 -> PX4 Landing Logic/6(MPC_LAND_ALT2_in)
  DSR_MPC_LAND_ALT3_const/1 -> PX4 Landing Logic/7(MPC_LAND_ALT3_in)
  PX4 Landing Logic/1(pos_sp) -> pos_sp/1
  PX4 Landing Logic/2(vel_sp) -> vel_sp/1
  PX4 Landing Logic/3(acc_sp) -> acc_sp/1
  land_trigger/1 -> PX4 Landing Logic/1(land_trigger)

== system flightControlSystem/SetpointManager/Simulation Set target Position/Setpoints Selector ==
  Land_Pos : Inport
  Land_Vel : Inport  Port=2
  Land_Acc : Inport  Port=3
  LandTrigger : Inport  Port=4
  Des_Pos : Inport  Port=5
  Des_Vel : Inport  Port=6
  Des_Acc : Inport  Port=7
  Acc Switch : Switch  Criteria=u2 > Threshold  SaturateOnIntegerOverflow=off  InputSameDT=off
  Rate Transition2 : RateTransition
  Rate Transition4 : RateTransition
  Rate Transition5 : RateTransition
  Reshape : Reshape
  Switch : Switch  Criteria=u2 > Threshold  SaturateOnIntegerOverflow=off  InputSameDT=off
  Vel Switch : Switch  Criteria=u2 > Threshold  SaturateOnIntegerOverflow=off  InputSameDT=off
  des_pos : Outport
  des_vel : Outport  Port=2
  des_acc : Outport  Port=3
  wires:
  Land_Acc/1 -> Acc Switch/1
  Acc Switch/1 -> Rate Transition5/1
  Reshape/1 -> Switch/1
  LandTrigger/1 -> Vel Switch/2, Switch/2, Acc Switch/2
  Switch/1 -> Rate Transition2/1
  Vel Switch/1 -> Rate Transition4/1
  Land_Pos/1 -> Reshape/1
  Land_Vel/1 -> Vel Switch/1
  Rate Transition2/1 -> des_pos/1
  Des_Pos/1 -> Switch/3
  Rate Transition4/1 -> des_vel/1
  Des_Vel/1 -> Vel Switch/3
  Rate Transition5/1 -> des_acc/1
  Des_Acc/1 -> Acc Switch/3

== system flightControlSystem/Actuator Commands/Simulation Actuator Commands/Mixer/Battery_Scaling ==
  In1 : Inport
  In2 : Inport  Port=2
  Compare To Constant : simulink/Logic and Bit Operations/Compare To Constant  relop=~=  const=0  OutDataTypeStr=boolean
  Constant : Constant  SampleTime=SampleTime
  Demux1 : Demux  Outputs=3
  Gain : Gain  Gain=-1
  Product : Product
  Product2 : Product
  Saturation1 : Saturate  UpperLimit=1  LowerLimit=-1
  Saturation2 : Saturate  UpperLimit=1  LowerLimit=-1
  Switch : Switch  Criteria=u2 > Threshold  SaturateOnIntegerOverflow=off  InputSameDT=off
  Switch1 : Switch  Criteria=u2 > Threshold  SaturateOnIntegerOverflow=off  InputSameDT=off
  thrust_setpoint : Outport
  pitch : Outport  Port=2
  roll : Outport  Port=3
  yaw : Outport  Port=4
  wires:
  Constant/1 -> Product2/2, Compare To Constant/1, Product/2  "<scale>"
  In1/1 -> Switch/3, Product/1
  In2/1 -> Switch1/3, Product2/1
  Switch/1 -> Gain/1
  Product/1 -> Switch/1
  Gain/1 -> Saturation2/1
  Demux1/3 -> yaw/1
  Switch1/1 -> Saturation1/1
  Compare To Constant/1 -> Switch1/2, Switch/2
  Saturation1/1 -> Demux1/1  "torque_setpoint"
  Product2/1 -> Switch1/1
  Demux1/1 -> roll/1
  Demux1/2 -> pitch/1
  Saturation2/1 -> thrust_setpoint/1  "thrust_setpoint"

== system flightControlSystem/MultiCopter Controller/Angular Rate Control/RateIntegral_State/Set target Position ==
  Control_Power : Inport
  Bus Assignment : BusAssignment  AssignedSignals=timestamp,control_power
  PX4 Timestamp : px4Utilslib/PX4 Timestamp  SampleTime=-1
  PX4 uORB Message : px4uORBlib/PX4 uORB Message  uORBMsg=ActuatorControlsStatus  uORBTopicName=actuator_controls_status_0  isSingleTopicMsg=off  SampleTime=-1
  PX4 uORB Write : px4uORBlib/PX4 uORB Write  uORBMsg=ActuatorControlsStatus  uORBTopicName=actuator_controls_status_0  PublishOption=None  OutputPublishedInstanceNum=off  selectInstanceNum=1  OutputStatus=off  isSingleTopicMsg=off
  wires:
  PX4 Timestamp/1 -> Bus Assignment/2
  PX4 uORB Message/1 -> Bus Assignment/1
  Bus Assignment/1 -> PX4 uORB Write/1
  Control_Power/1 -> Bus Assignment/3

== system flightControlSystem/MultiCopter Controller/Angular Rate Control/RateIntegral_State/Simulation Set target Position ==
  Control_Power : Inport
  Terminator3 : Terminator
  wires:
  Control_Power/1 -> Terminator3/1

== system flightControlSystem/MultiCopter Controller/Angular Rate Control/RatePID_Core/ActuatorSaturation_Detector ==
  unallocated_torque_3x1 : Inport
  torque_setpoint_achieved : Inport  Port=2
  If Action Subsystem1 : Subsystem  TreatAsAtomicUnit=on
  If1 : If  IfExpression=u1 ~= 0
  Merge1 : Merge
  Merge2 : Merge
  NOT1 : Logic  Operator=NOT  IconShape=distinctive  AllPortsSameDT=off  OutDataTypeStr=boolean
  Subsystem1 : Subsystem
  is_saturated_positive_3x1 : Outport
  is_saturated_negative_3x1 : Outport  Port=2
  wires:
  If Action Subsystem1/2(saturation_negative) -> Merge2/2
  Merge1/1 -> is_saturated_positive_3x1/1
  If Action Subsystem1/1(saturation_positive) -> Merge1/2
  If1/2 -> If Action Subsystem1/Action
  Subsystem1/2(saturation_negative) -> Merge2/1
  If1/1 -> Subsystem1/Action
  NOT1/1 -> If1/1
  Subsystem1/1(saturation_positive) -> Merge1/1
  torque_setpoint_achieved/1 -> NOT1/1
  unallocated_torque_3x1/1 -> Subsystem1/1(unallocated_torque)
  Merge2/1 -> is_saturated_negative_3x1/1

== system flightControlSystem/MultiCopter Controller/Angular Rate Control/RatePID_Core/rate_integral ==
  mixer_saturated_positive : Inport
  mixer_saturated_negative : Inport  Port=2
  gain_I_per_axis : Inport  Port=3
  landed_reset_to_zero : Inport  Port=4
  airborne_update_integral : Inport  Port=5
  integral_limit_symmetric : Inport  Port=6
  dt_s : Inport  Port=7
  rate_error_rads : Inport  Port=8
  integral_state_previous : Inport  Port=9
  AntiWindup_IntegralUpdate : Subsystem
  IfLanded_ResetIntegral_PassZero : Subsystem  TreatAsAtomicUnit=on
  Merge : Merge
  integral_state_updated : Outport
  wires:
  IfLanded_ResetIntegral_PassZero/1(Out1) -> Merge/2
  mixer_saturated_positive/1 -> AntiWindup_IntegralUpdate/1(is_saturated_positive_3x1)
  landed_reset_to_zero/1 -> AntiWindup_IntegralUpdate/Action
  integral_limit_symmetric/1 -> AntiWindup_IntegralUpdate/4(integral_limit_symmetric)
  dt_s/1 -> AntiWindup_IntegralUpdate/7(dt_s)
  AntiWindup_IntegralUpdate/1(integral_state_new) -> Merge/1
  mixer_saturated_negative/1 -> AntiWindup_IntegralUpdate/2(is_saturated_negative_3x1)
  integral_state_previous/1 -> AntiWindup_IntegralUpdate/6(integral_state_prev), IfLanded_ResetIntegral_PassZero/1(rate_int_in)
  Merge/1 -> integral_state_updated/1
  gain_I_per_axis/1 -> AntiWindup_IntegralUpdate/3(gain_I_per_axis)
  rate_error_rads/1 -> AntiWindup_IntegralUpdate/5(rate_error_rads)
  airborne_update_integral/1 -> IfLanded_ResetIntegral_PassZero/Action

== system flightControlSystem/MultiCopter Controller/Attitude_Controller/AttitudeControl/vectorToQuaternion ==
  z_axis_unit_vector : Inport
  desired_z_axis_from_qd : Inport  Port=2
  Cast To Double : DataTypeConversion  OutDataTypeStr=double  SaturateOnIntegerOverflow=off  RndMeth=Floor
  MATLAB Function : MATLAB Function  TreatAsAtomicUnit=on
  Normalize Vector : vrlib/Utilities/Normalize Vector  maxzero=0
  q_tilt_rotation : Outport
  wires:
  z_axis_unit_vector/1 -> MATLAB Function/1(src)
  desired_z_axis_from_qd/1 -> MATLAB Function/2(dst)
  MATLAB Function/1(q) -> Cast To Double/1
  Normalize Vector/1 -> q_tilt_rotation/1
  Cast To Double/1 -> Normalize Vector/1

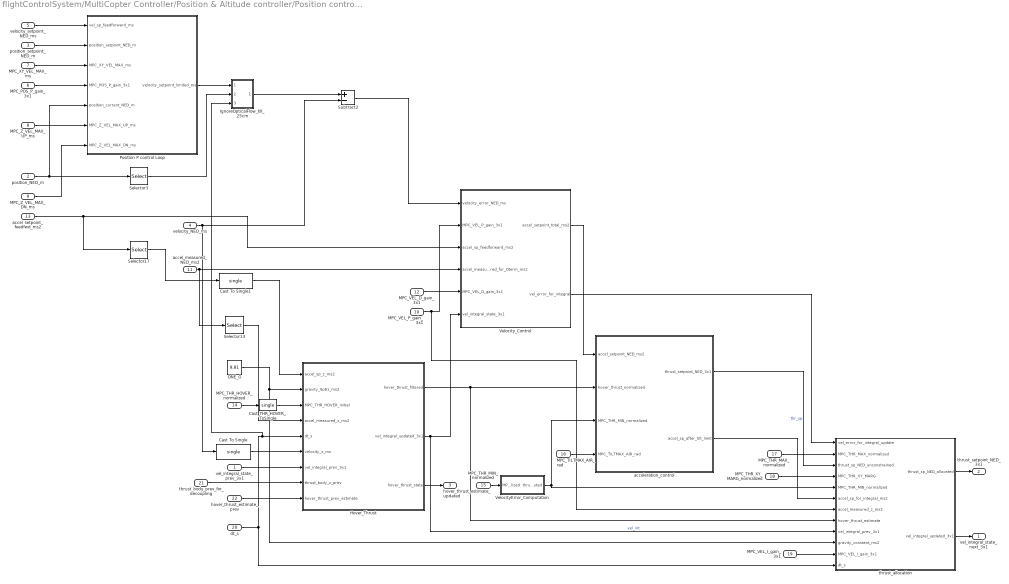
== system flightControlSystem/MultiCopter Controller/Position & Altitude controller/Position controller/PositionVelocityControl ==
  vel_integral_state_prev_3x1 : Inport
  position_NED_m : Inport  Port=2
  position_setpoint_NED_m : Inport  Port=3
  velocity_NED_ms : Inport  Port=4
  velocity_setpoint_NED_ms : Inport  Port=5
  MPC_POS_P_gain_3x1 : Inport  Port=6
  MPC_XY_VEL_MAX_ms : Inport  Port=7
  MPC_Z_VEL_MAX_UP_ms : Inport  Port=8
  MPC_Z_VEL_MAX_DN_ms : Inport  Port=9
  MPC_VEL_P_gain_3x1 : Inport  Port=10
  accel_measured_NED_ms2 : Inport  Port=11
  MPC_VEL_D_gain_3x1 : Inport  Port=12
  accel_setpoint_feedfwd_ms2 : Inport  Port=13
  MPC_THR_HOVER_normalized : Inport  Port=14
  MPC_THR_MIN_normalized : Inport  Port=15
  MPC_TILTMAX_AIR_rad : Inport  Port=16
  MPC_THR_MAX_normalized : Inport  Port=17
  MPC_THR_XY_MARG_normalized : Inport  Port=18
  MPC_VEL_I_gain_3x1 : Inport  Port=19
  dt_s : Inport  Port=20
  thrust_body_prev_for_decoupling : Inport  Port=21
  hover_thrust_estimate_prev : Inport  Port=22
  Cast To Single : DataTypeConversion  OutDataTypeStr=single  SaturateOnIntegerOverflow=off  RndMeth=Floor
  Cast To Single1 : DataTypeConversion  OutDataTypeStr=single  SaturateOnIntegerOverflow=off  RndMeth=Floor
  Cast_THR_HOVER_ToSingle : DataTypeConversion  OutDataTypeStr=single  SaturateOnIntegerOverflow=off  RndMeth=Floor
  Hover_Thrust : Subsystem
  IgnoreOpticalFlow_till_25cm : Subsystem
  ONE_G : Constant  Value=9.81  OutDataTypeStr=single  SampleTime=-1
  Position P control Loop : Subsystem
  Selector13 : Selector  InputPortWidth=3  IndexOptions=Index vector (dialog)  Indices=3  OutputSizes=1  RuntimeRangeChecks=off
  Selector17 : Selector  InputPortWidth=3  IndexOptions=Index vector (dialog)  Indices=3  OutputSizes=1  RuntimeRangeChecks=off
  Selector3 : Selector  InputPortWidth=3  IndexOptions=Index vector (dialog)  Indices=[3]  OutputSizes=1  RuntimeRangeChecks=off
  Subtract2 : Sum  Inputs=+-
  VelocityError_Computation : Subsystem
  Velocity_Control : Subsystem
  acceleration_control : Subsystem
  thrust_allocation : Subsystem
  vel_integral_state_next_3x1 : Outport
  thrust_setpoint_NED_3x1 : Outport  Port=2
  hover_thrust_estimate_updated : Outport  Port=3
  wires:
  accel_setpoint_feedfwd_ms2/1 -> Velocity_Control/3(accel_sp_feedforward_ms2), Selector17/1
  velocity_setpoint_NED_ms/1 -> Position P control Loop/1(vel_sp_feedforward_ms)
  position_setpoint_NED_m/1 -> Position P control Loop/2(position_setpoint_NED_m)
  position_NED_m/1 -> Selector3/1, Position P control Loop/5(position_current_NED_m)
  MPC_XY_VEL_MAX_ms/1 -> Position P control Loop/3(MPC_XY_VEL_MAX_ms)
  MPC_POS_P_gain_3x1/1 -> Position P control Loop/4(MPC_POS_P_gain_3x1)
  MPC_Z_VEL_MAX_UP_ms/1 -> Position P control Loop/6(MPC_Z_VEL_MAX_UP_ms)
  MPC_Z_VEL_MAX_DN_ms/1 -> Position P control Loop/7(MPC_Z_VEL_MAX_DN_ms)
  Position P control Loop/1(velocity_setpoint_limited_ms) -> IgnoreOpticalFlow_till_25cm/1(velocity_from_optical_flow)
  accel_measured_NED_ms2/1 -> Velocity_Control/4(accel_measured_for_Dterm_ms2), Selector13/1
  Selector3/1 -> IgnoreOpticalFlow_till_25cm/2(altitude_AGL_m)
  velocity_NED_ms/1 -> Cast To Single/1, Subtract2/2
  Selector17/1 -> Cast To Single1/1
  IgnoreOpticalFlow_till_25cm/1(velocity_flow_gated) -> Subtract2/1
  Cast To Single1/1 -> Hover_Thrust/1(accel_sp_z_ms2)
  Selector13/1 -> Hover_Thrust/4(accel_measured_z_ms2)
  ONE_G/1 -> thrust_allocation/10(gravity_constant_ms2), Hover_Thrust/2(gravity_9p81_ms2)
  Cast To Single/1 -> Hover_Thrust/6(velocity_z_ms)
  vel_integral_state_prev_3x1/1 -> Hover_Thrust/7(vel_integral_prev_3x1)
  dt_s/1 -> IgnoreOpticalFlow_till_25cm/3(dt_s), Hover_Thrust/5(dt_s), thrust_allocation/12(dt_s)
  thrust_body_prev_for_decoupling/1 -> Hover_Thrust/8(thrust_body_z_prev)
  hover_thrust_estimate_prev/1 -> Hover_Thrust/9(hover_thrust_prev_estimate)
  Subtract2/1 -> Velocity_Control/1(velocity_error_NED_ms)
  MPC_VEL_D_gain_3x1/1 -> Velocity_Control/5(MPC_VEL_D_gain_3x1)
  MPC_VEL_P_gain_3x1/1 -> thrust_allocation/7(accel_measured_z_ms2), Velocity_Control/2(MPC_VEL_P_gain_3x1)
  MPC_THR_MIN_normalized/1 -> VelocityError_Computation/1(MPC_THR_MIN_normalized)
  thrust_allocation/1(thrust_sp_NED_allocated) -> thrust_setpoint_NED_3x1/1
  MPC_TILTMAX_AIR_rad/1 -> acceleration_control/4(MPC_TILTMAX_AIR_rad)
  Hover_Thrust/2(vel_integral_updated_3x1) -> thrust_allocation/9(vel_integral_prev_3x1), Velocity_Control/6(vel_integral_state_3x1)  "vel_int"
  Hover_Thrust/1(hover_thrust_filtered) -> thrust_allocation/8(hover_thrust_estimate), acceleration_control/2(hover_thrust_normalized)
  Hover_Thrust/3(hover_thrust_state) -> hover_thrust_estimate_updated/1
  Velocity_Control/2(vel_error_for_integral) -> thrust_allocation/1(vel_error_for_integral_update)
  Velocity_Control/1(accel_setpoint_total_ms2) -> acceleration_control/1(accel_setpoint_NED_ms2)
  VelocityError_Computation/1(thrust_min_adjusted) -> acceleration_control/3(MPC_THR_MIN_normalized), thrust_allocation/5(MPC_THR_MIN_normalized)
  MPC_THR_MAX_normalized/1 -> thrust_allocation/2(MPC_THR_MAX_normalized)
  MPC_THR_XY_MARG_normalized/1 -> thrust_allocation/4(MPC_THR_XY_MARG)
  acceleration_control/2(accel_sp_after_tilt_limit) -> thrust_allocation/6(accel_sp_for_integral_ms2)
  acceleration_control/1(thrust_setpoint_NED_3x1) -> thrust_allocation/3(thrust_sp_NED_unconstrained)  "thr_sp"
  MPC_VEL_I_gain_3x1/1 -> thrust_allocation/11(MPC_VEL_I_gain_3x1)
  thrust_allocation/2(vel_integral_updated_3x1) -> vel_integral_state_next_3x1/1
  MPC_THR_HOVER_normalized/1 -> Cast_THR_HOVER_ToSingle/1
  Cast_THR_HOVER_ToSingle/1 -> Hover_Thrust/3(MPC_THR_HOVER_initial)
